simulink model "AXU5EV_Experiment_Duty_HDL"  (R2026b)
settings: Solver=FixedStepDiscrete  StopTime=0.000001  FixedStep=2e-8
settings Model: Creator=lww  LastModifiedBy=lww

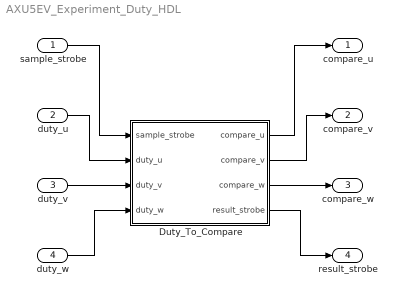
== system AXU5EV_Experiment_Duty_HDL ==
  sample_strobe : Inport  OutDataTypeStr=boolean  SampleTime=2e-8
  duty_u : Inport  Port=2  OutDataTypeStr=uint32  SampleTime=2e-8
  duty_v : Inport  Port=3  OutDataTypeStr=uint32  SampleTime=2e-8
  duty_w : Inport  Port=4  OutDataTypeStr=uint32  SampleTime=2e-8
  Duty_To_Compare : Subsystem
  compare_u : Outport
  compare_v : Outport  Port=2
  compare_w : Outport  Port=3
  result_strobe : Outport  Port=4
  wires:
  Duty_To_Compare/4(result_strobe) -> result_strobe/1
  duty_w/1 -> Duty_To_Compare/4(duty_w)
  Duty_To_Compare/3(compare_w) -> compare_w/1
  duty_v/1 -> Duty_To_Compare/3(duty_v)
  Duty_To_Compare/2(compare_v) -> compare_v/1
  duty_u/1 -> Duty_To_Compare/2(duty_u)
  Duty_To_Compare/1(compare_u) -> compare_u/1
  sample_strobe/1 -> Duty_To_Compare/1(sample_strobe)

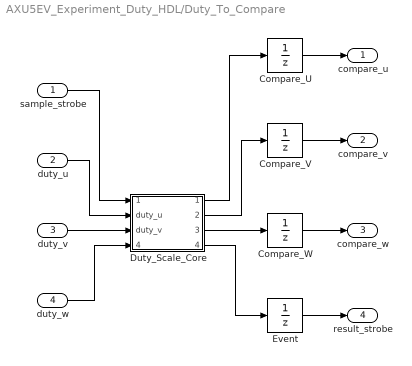
== system AXU5EV_Experiment_Duty_HDL/Duty_To_Compare ==
  sample_strobe : Inport  OutDataTypeStr=boolean  SampleTime=2e-8
  duty_u : Inport  Port=2  OutDataTypeStr=uint32  SampleTime=2e-8
  duty_v : Inport  Port=3  OutDataTypeStr=uint32  SampleTime=2e-8
  duty_w : Inport  Port=4  OutDataTypeStr=uint32  SampleTime=2e-8
  Compare_U : UnitDelay  SampleTime=-1
  Compare_V : UnitDelay  SampleTime=-1
  Compare_W : UnitDelay  SampleTime=-1
  Duty_Scale_Core : MATLAB Function  TreatAsAtomicUnit=on
  Event : UnitDelay  SampleTime=-1
  compare_u : Outport
  compare_v : Outport  Port=2
  compare_w : Outport  Port=3
  result_strobe : Outport  Port=4
  wires:
  Event/1 -> result_strobe/1
  Compare_W/1 -> compare_w/1
  Compare_V/1 -> compare_v/1
  Compare_U/1 -> compare_u/1
  Duty_Scale_Core/4(result_strobe) -> Event/1
  Duty_Scale_Core/3(compare_w) -> Compare_W/1
  Duty_Scale_Core/2(compare_v) -> Compare_V/1
  Duty_Scale_Core/1(compare_u) -> Compare_U/1
  duty_w/1 -> Duty_Scale_Core/4(duty_w)
  duty_v/1 -> Duty_Scale_Core/3(duty_v)
  duty_u/1 -> Duty_Scale_Core/2(duty_u)
  sample_strobe/1 -> Duty_Scale_Core/1(sample_strobe)

== matlab function AXU5EV_Experiment_Duty_HDL/Duty_To_Compare/Duty_Scale_Core ==
  data: sample_strobe input; compare_u output; duty_u input; duty_v input; duty_w input; compare_v output; compare_w output; result_strobe output
function [compare_u,compare_v,compare_w,result_strobe]=f(sample_strobe,duty_u,duty_v,duty_w)
[compare_u,compare_v,compare_w,result_strobe]=axu5ev_experiment_duty_to_compare(sample_strobe,duty_u,duty_v,duty_w);
end
